simulink model "controller"  (Simulink 7.0)
settings: Solver=FixedStepDiscrete  StartTime=0.0  StopTime=10.0  FixedStep=0.03  RelTol=1e-3
undefined symbols (not defined in the file or in its folder): OC1max
libraries: dsPICdrivers x7
settings Model: Creator=zhaosy  LastModifiedBy=zhaosy
settings OptimizationCC: OptimizeModelRefInitCode=on  LifeSpan=1
settings HardwareCC: ProdBitPerInt=16  ProdEndianess=LittleEndian  ProdWordSize=16  ProdHWDeviceType=16-bit Generic  TargetHWDeviceType=32-bit Generic
settings RTWCC: SystemTargetFile=dspic.tlc  TemplateMakefile=dspic_pic30_gcc.tmf  PostCodeGenCommand=dsPIC_Compile()  Description=Embedded Target for Microchip dsPIC (real-time)  ProcessScript=dspic_make_rtw_hook
settings CodeAppCC: IgnoreCustomStorageClasses=off
settings STFCustomTargetCC: GenFloatMathFcnCalls=ANSI_C  ModelReferenceCompliant=off  IncludeMdlTerminateFcn=off  CombineOutputUpdateFcns=on  SuppressErrorStatus=on  ERTCustomFileBanners=on  SupportContinuousTime=off  SupportNonInlinedSFcns=off  SystemTargetFile=dspic.tlc
settings ERTTargetCC: GenFloatMathFcnCalls=ANSI_C  ModelReferenceCompliant=off  CompOptLevelCompliant=off  IncludeMdlTerminateFcn=off  SuppressErrorStatus=on  ModelStepFunctionPrototypeControlCompliant=off  InlinedParameterPlacement=NonHierarchical  ERTSrcFileBannerTemplate=dsPIC_code_template.cgt  ERTHdrFileBannerTemplate=dsPIC_code_template.cgt  ERTDataSrcFileTemplate=dsPIC_code_template.cgt  ERTDataHdrFileTemplate=dsPIC_code_template.cgt  ERTCustomFileTemplate=dsPIC_main.tlc
settings CustomProperty: DataType=string  Value=C:\MATLAB\R2007b\bin\win32\gmake

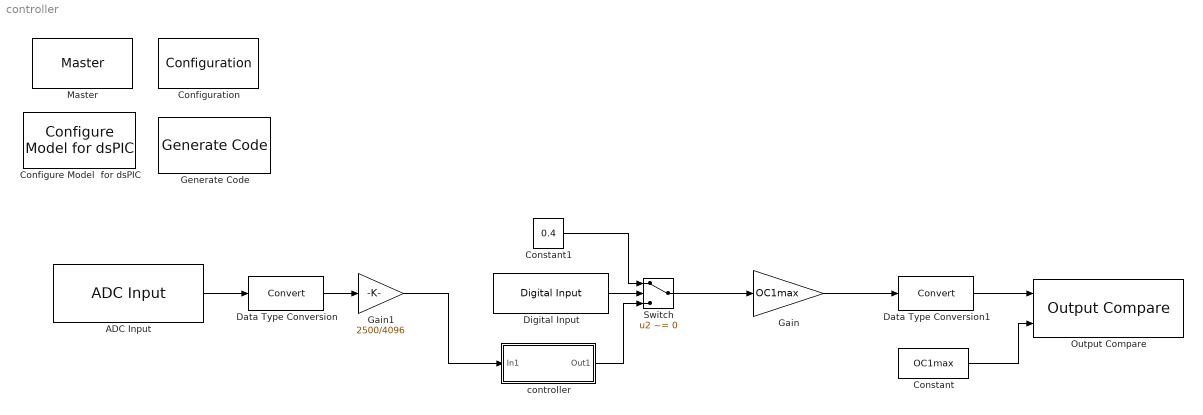
== system controller ==
  ADC Input : dsPICdrivers/Peripheral I//O/ADC Input  Tag=dsPIC_ADC  Priority=5  ADC_TYPE=12 bits  ADC_MODE=Continuous sampling & get last channel value  NbrSampleStep=1  VoltRefpopup="AVdd  -  AVss"  OutFormatBitspopup=0000 dddd dddd dddd : Integer  InterruptPriority=6  ANCHANNELS=[6]  MaxName=ANmax = 4096  Rin=5000  ADCS=19  SAMC=1  Temperature=15  DMAChannel=0  SampleTime=-1  Status="OK  |  Tsmp=6.782e-007 |  T/Channel=1.017e-005 |  Tall=1.017e-005"
  Configuration : dsPICdrivers/Configuration  SystemSampleTime=-1  double64=on
  Configure Model  for dsPIC : dsPICdrivers/Simulink Configuration/Configure Model  for dsPIC
  Constant : Constant  Value=OC1max  OutDataTypeMode=uint16  OutDataType=sfix(16)  OutScaling=2^0  SampleTime=-1
  Constant1 : Constant  Value=0.4  OutDataTypeMode=double  OutDataType=sfix(16)  OutScaling=2^0  SampleTime=-1
  Data Type Conversion : DataTypeConversion  OutDataTypeMode=double  OutDataType=sfix(16)  OutScaling=2^0
  Data Type Conversion1 : DataTypeConversion  OutDataTypeMode=uint16  OutDataType=sfix(16)  OutScaling=2^0
  Digital Input : dsPICdrivers/Digital I//O/Digital Input  Tag=dsPIC_Digital_Input  PORT=A  Pin=[12]  SampleTime=-1  OrderingInOutPopup=None
  Gain : Gain  Gain=OC1max  ParameterDataTypeMode=double  ParameterDataType=sfix(16)  ParameterScaling=2^0  OutDataTypeMode=double  OutDataType=sfix(16)  OutScaling=2^0
  Gain1 : Gain  Gain=2500/4096  ParameterDataTypeMode=double  ParameterDataType=sfix(16)  ParameterScaling=2^0  OutDataTypeMode=double  OutDataType=sfix(16)  OutScaling=2^0
  Generate Code : dsPICdrivers/Simulink Configuration/Generate Code
  Master : dsPICdrivers/Master  Tag=dsPIC_MASTER  Priority=1  TimeStepType=Timer1  picType=30f6014A  fcy=14745600  Quartz_33f=5e6  PLLActive_33f=off  fcyDesired_33f=0  tmr1="[8  55295  0]"  tmr1Info="Time Step : 0.03  ;   Error : 0%  PR1=55295"  tmr2345="[1  0  0  0]"  tmr2345cfg=[-1 -1 -1 -1]  IOautoConf=on  typePort="[ 0  0  0  0  0  0  0  0  0  0  0  0  9  0  0  0  0  0  0  0  0  0  8  0  0  0  0  0  0  0  0  0  0  0  0  0  0  0  0  0  0  0  0  0  0  0  0  0  7  0  0  0  0  0  0  0  0  0  0  0  0  0  0  0  0  0  0  0  0  0  0  0  0  0  0  0  0  0  0  0  0  0  0  0  0  0  0  0  0  0  0  0  0  0  0  0  0  0  0  0  0  0  0  0  0  0  0  0  0  0  0  0 ]"  TRIS="[ 65535  65535  65535  65534  65535  65535  65535 ]"  ADPCFG=0  MasterBusyPort=None  MasterOverloadPort=None  FOSC=XT_PLL8  ClockSwitchMonitor=Both disabled  TempProtection_33f=TEMP_ON  FPBOR=PBOR_OFF  PWRT=PWRT_OFF  MCLR=MCLR_DIS  PowerSave=off  OverrideFcy=off  NewFcy=1e6
  Output Compare : dsPICdrivers/Peripheral I//O/Output Compare  Tag=dsPIC_PWM_out  Priority=5  IntPriority=3  CHANNEL=[1]  Channel_UP_Down_Periode=[5]  MaxChannel=[0.0033]  MaxName=' OC1max '  Precision=[15.5705]  Timer=[2]  Status=OK  SafeMarge=[0]  PortLetter=[68]  PortNumber=[0]  MaxValues=[48660.48]
  Switch : Switch  Criteria=u2 ~= 0  OutDataTypeMode=double  OutDataType=sfix(16)  OutScaling=2^0
  controller : Subsystem  TreatAsAtomicUnit=on
  wires:
  Constant/1 -> Output Compare/2
  Gain/1 -> Data Type Conversion1/1
  Switch/1 -> Gain/1
  Data Type Conversion/1 -> Gain1/1
  Gain1/1 -> controller/1(In1)
  Data Type Conversion1/1 -> Output Compare/1
  Digital Input/1 -> Switch/2
  controller/1(Out1) -> Switch/3
  Constant1/1 -> Switch/1
  ADC Input/1 -> Data Type Conversion/1

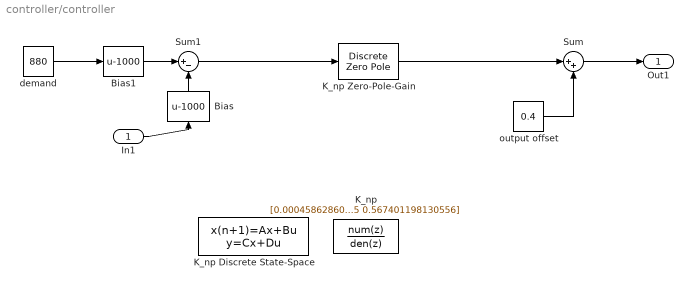
== system controller/controller ==
  In1 : Inport
  Bias : Bias  Orientation=up  Bias=-1000
  Bias1 : Bias  Bias=-1000
  K_np : DiscreteTransferFcn  Numerator="[0.000458628605161927\t-0.00258407315341432\t0.00605666798625169\t-0.00755785286680422\t0.00529486332815921\t-0.00197424578940870\t0.000306011890280094]"  Denominator="[1\t-5.51488039636196\t12.6275299975999\t-15.3607039992067\t10.4657408046876\t-3.78508760484525\t0.567401198130556]"  SampleTime=-1
  K_np Discrete State-Space : DiscreteStateSpace  A=|  B=|  C="[-0.00350663997414266\t0.00424514426899289\t-0.00410395693874253\t0.00395980176735258\t-0.00190637072626259\t0.00146513504685667]"  D=4.586286051619270e-04  SampleTime=-1
      A=|
      | [5.51488039636196	-3.15688249939998	1.92008799990084	-1.30821760058595	0.473135950605656	-0.283700599065278; 4	0	0	0	0	0;
      | 0	2	0	0	0	0;
      | 0	0	1	0	0	0;
      | 0	0	0	1	0	0;
      | 0	0	0	0	0.25 0]
      B=|
      | [0.015625;
      | 0;
      | 0;
      | 0;
      | 0;
      | 0]
  K_np Zero-Pole-Gain : DiscreteZeroPole  Zeros=|  Poles=|  Gain=4.586286051619270e-04  SampleTime=-1
      Zeros=|
      | [0.993200209674043+0.00585031974890255i
      | 0.993200209674043-0.00585031974890255i
      | 0.992415356351071+0.00000000000000i
      | 0.952832144799046+0.0316012985820410i
      | 0.952832144799046-0.0316012985820410i
      | 0.749867911105068+0.00000000000000i]
      Poles=|
      | [0.996570824147705+0.00712395634689976i
      | 0.996570824147705-0.00712395634689976i
      | 0.999707020427791+0.00000000000000i
      | 0.995227816713482+0.00000000000000i
      | 0.856091901895871+0.00000000000000i
      | 0.670712009029412+0.00000000000000i]
  Sum : Sum  Inputs=|++  OutDataTypeMode=double  OutDataType=fixdt(1,16,6)
  Sum1 : Sum  Inputs=|+-  OutDataTypeMode=double  OutDataType=fixdt(1,16,3)
  demand : Constant  Value=880  VectorParams1D=off  OutDataTypeMode=double  OutDataType=fixdt(1,16,3)  ConRadixGroup=Best Precision: Vector-wise  SampleTime=-1
  output offset : Constant  Value=0.4  VectorParams1D=off  OutDataTypeMode=double  OutDataType=fixdt(1,16,6)  ConRadixGroup=Best Precision: Vector-wise  SampleTime=-1
  Out1 : Outport  OutDataType=sfix(16)  OutScaling=2^0
  wires:
  Sum/1 -> Out1/1
  output offset/1 -> Sum/2
  Bias1/1 -> Sum1/1
  Bias/1 -> Sum1/2
  Sum1/1 -> K_np Zero-Pole-Gain/1
  In1/1 -> Bias/1
  demand/1 -> Bias1/1
  K_np Zero-Pole-Gain/1 -> Sum/1
